simulink model "fix_Current_sync"  (R2025b)
settings: Solver=FixedStepAuto  StartTime=0.0  StopTime=20  FixedStep=0.001  RelTol=1e-3
values from neighbouring files (symbols this model uses):
  Dm = 1e-3    (= 0.001)    [motor_param.m]
  Ki_s = 0.041    [motor_param.m]
  Kp_s = 0.0014    [motor_param.m]
  Ld = 0.01    [motor_param.m]
  Lq = 0.02    [motor_param.m]
  p = 2    [motor_param.m]
  Phi = 0.1    [motor_param.m]
  Rs = 0.38    [motor_param.m]
libraries: fl_lib x50, nesl_utility x50, ee_lib x15, eeTransforms x10, slpidlib x5
(part 1 of 3)
settings Model: Creator=ZhiyongXu  LastModifiedBy=ZhiyongXu

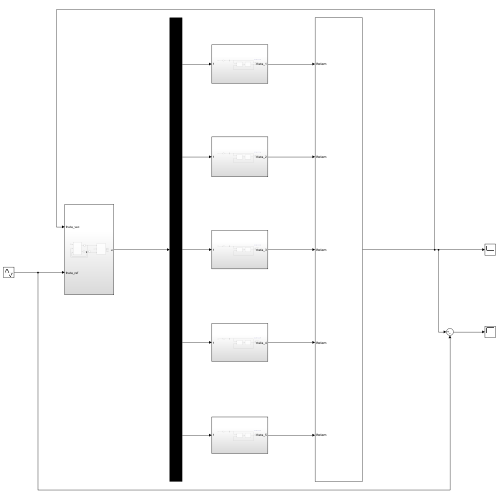
[thumbnail: Simulink's stored preview of the top-level diagram]
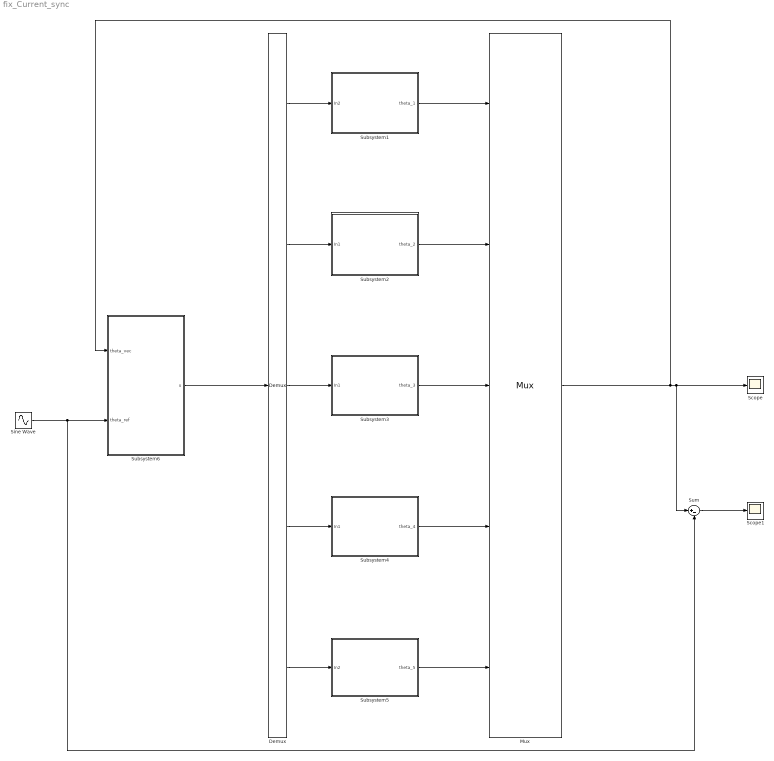
== system fix_Current_sync ==
  Demux : Demux  Outputs=5
  Mux : Mux  Inputs=5
      settings: DisplayOption=signals
  Scope : Scope
      settings: ActiveDisplayYMinimum=-15.273107398212424  ActiveDisplayYMaximum=29.223277886779115  DataLoggingVariableName=ScopeData2  DataLoggingSaveFormat=Array
  Scope1 : Scope
      settings: ActiveDisplayYMinimum=-22.387708842916332  ActiveDisplayYMaximum=22.665034162770731  DataLoggingVariableName=ScopeData3
  Sine Wave : Sin  Amplitude=10  SampleTime=0
  Subsystem1 : Subsystem
  Subsystem2 : Subsystem
  Subsystem3 : Subsystem
  Subsystem4 : Subsystem
  Subsystem5 : Subsystem
  Subsystem6 : Subsystem
  Sum : Sum  Inputs=|+-
  wires:
  Sine Wave/1 -> Sum/2, Subsystem6/2(theta_ref)
  Subsystem6/1(u) -> Demux/1
  Demux/1 -> Subsystem1/1(In2)
  Demux/2 -> Subsystem2/1(In1)
  Demux/3 -> Subsystem3/1(In1)
  Demux/4 -> Subsystem4/1(In1)
  Subsystem1/1(theta_1) -> Mux/1
  Subsystem2/1(theta_2) -> Mux/2
  Subsystem3/1(theta_3) -> Mux/3
  Subsystem4/1(theta_4) -> Mux/4
  Subsystem5/1(theta_5) -> Mux/5
  Sum/1 -> Scope1/1
  Mux/1 -> Sum/1, Scope/1, Subsystem6/1(theta_vec)
  Demux/5 -> Subsystem5/1(In2)

== system fix_Current_sync/Subsystem1 ==
  note: Tune the PI gains of velocity controller
  note: Final Values
  note: Start Values
  In2 : Inport
  Bus Creator : BusCreator  Inputs=1
  Controller : Subsystem
  Evaluation : Subsystem
  Plant : Subsystem
  rpm2rads : Gain
  theta_1 : Outport
  wires:
  Evaluation/1(Out1) -> theta_1/1
  Plant/1(MeasSigs) -> Evaluation/2(MeasSigs), Controller/2(MeasSigs)
  Controller/1(MotCmds) -> Plant/1(MotCmds)
  Bus Creator/1 -> Evaluation/1(TestSigs), Controller/1(TestSigs)
  In2/1 -> rpm2rads/1
  rpm2rads/1 -> Bus Creator/1  "wmref"

== system fix_Current_sync/Subsystem2 ==
  note: Tune the PI gains of velocity controller
  note: Final Values
  note: Start Values
  In1 : Inport
  Bus Creator : BusCreator  Inputs=1
  Controller : Subsystem
  Evaluation : Subsystem
  Plant : Subsystem
  rpm2rads : Gain
  theta_2 : Outport
  wires:
  Evaluation/1(Out1) -> theta_2/1
  Plant/1(MeasSigs) -> Evaluation/2(MeasSigs), Controller/2(MeasSigs)
  Controller/1(MotCmds) -> Plant/1(MotCmds)
  Bus Creator/1 -> Evaluation/1(TestSigs), Controller/1(TestSigs)
  In1/1 -> rpm2rads/1
  rpm2rads/1 -> Bus Creator/1  "wmref"

== system fix_Current_sync/Subsystem3 ==
  note: Tune the PI gains of velocity controller
  note: Final Values
  note: Start Values
  In1 : Inport
  Bus Creator : BusCreator  Inputs=1
  Controller : Subsystem
  Evaluation : Subsystem
  Plant : Subsystem
  rpm2rads : Gain
  theta_3 : Outport
  wires:
  Evaluation/1(Out1) -> theta_3/1
  Plant/1(MeasSigs) -> Evaluation/2(MeasSigs), Controller/2(MeasSigs)
  Controller/1(MotCmds) -> Plant/1(MotCmds)
  Bus Creator/1 -> Evaluation/1(TestSigs), Controller/1(TestSigs)
  rpm2rads/1 -> Bus Creator/1  "wmref"
  In1/1 -> rpm2rads/1

== system fix_Current_sync/Subsystem4 ==
  note: Tune the PI gains of velocity controller
  note: Final Values
  note: Start Values
  In1 : Inport
  Bus Creator : BusCreator  Inputs=1
  Controller : Subsystem
  Evaluation : Subsystem
  Plant : Subsystem
  rpm2rads : Gain
  theta_4 : Outport
  wires:
  Evaluation/1(Out1) -> theta_4/1
  Plant/1(MeasSigs) -> Evaluation/2(MeasSigs), Controller/2(MeasSigs)
  Controller/1(MotCmds) -> Plant/1(MotCmds)
  Bus Creator/1 -> Evaluation/1(TestSigs), Controller/1(TestSigs)
  rpm2rads/1 -> Bus Creator/1  "wmref"
  In1/1 -> rpm2rads/1

== system fix_Current_sync/Subsystem5 ==
  note: Tune the PI gains of velocity controller
  note: Final Values
  note: Start Values
  In2 : Inport
  Bus Creator : BusCreator  Inputs=1
  Controller : Subsystem
  Evaluation : Subsystem
  Plant : Subsystem
  rpm2rads : Gain
  theta_5 : Outport
  wires:
  Evaluation/1(Out1) -> theta_5/1
  Plant/1(MeasSigs) -> Evaluation/2(MeasSigs), Controller/2(MeasSigs)
  Controller/1(MotCmds) -> Plant/1(MotCmds)
  Bus Creator/1 -> Evaluation/1(TestSigs), Controller/1(TestSigs)
  In2/1 -> rpm2rads/1
  rpm2rads/1 -> Bus Creator/1  "wmref"

== system fix_Current_sync/Subsystem6 ==
  theta_vec : Inport
  theta_ref : Inport  Port=2
  Integrator : Integrator
  Integrator1 : Integrator
  MATLAB Function : MATLAB Function  TreatAsAtomicUnit=on
  MATLAB Function4 : MATLAB Function  TreatAsAtomicUnit=on
  Scope : Scope
      settings: ActiveDisplayYMinimum=-6624.1594678331894  ActiveDisplayYMaximum=6466.1304904081144  DataLoggingVariableName=ScopeData4
  Scope1 : Scope
      settings: ActiveDisplayYMinimum=-12.471784481812829  ActiveDisplayYMaximum=55.255314336175005  DataLoggingVariableName=ScopeData5
  u : Outport
  wires:
  MATLAB Function4/1(dth_hat) -> Integrator/1
  MATLAB Function4/2(dom_hat) -> Integrator1/1
  theta_vec/1 -> MATLAB Function/2(theta_meas)
  theta_ref/1 -> MATLAB Function4/1(theta0)
  Integrator1/1 -> Scope1/1, MATLAB Function4/3(om_hat), MATLAB Function/3(om_hat)
  Integrator/1 -> MATLAB Function/1(theta0), MATLAB Function4/2(th_hat)
  MATLAB Function/1(omega_cmd) -> u/1, Scope/1

== system fix_Current_sync/Subsystem1/Controller ==
  TestSigs : Inport
  MeasSigs : Inport  Port=2
  DriverPeripherals : Subsystem
  FOC : Subsystem
  SensorPeripherals : Subsystem
  TestChannel : Subsystem
  MotCmds : Outport  VectorParamsAs1DForOutWhenUnconnected=off
  wires:
  FOC/1(Vabc) -> DriverPeripherals/1(Vabc)
  DriverPeripherals/1(MotCmds) -> MotCmds/1
  TestSigs/1 -> TestChannel/1(TestSigs)
  TestChannel/1(wmref) -> FOC/1(wmref)
  MeasSigs/1 -> SensorPeripherals/1(MeasSigs)
  SensorPeripherals/1(wm) -> FOC/2(wm)
  SensorPeripherals/2(Iabc) -> FOC/3(Iabc)
  SensorPeripherals/3(thetam) -> FOC/4(thetam)

== system fix_Current_sync/Subsystem1/Evaluation ==
  TestSigs : Inport
  MeasSigs : Inport  Port=2
  Bus Selector : BusSelector  OutputSignals=wmref
  Bus Selector1 : BusSelector  OutputSignals=wm,thetam
  Mux : Mux  Inputs=2
  Scope : Scope
      settings: ActiveDisplayYMinimum=-145.10741516627655  ActiveDisplayYMaximum=117.27907525237589
  rads2rpm : Gain
  Out1 : Outport
  wires:
  TestSigs/1 -> Bus Selector/1
  Mux/1 -> rads2rpm/1
  rads2rpm/1 -> Scope/1
  MeasSigs/1 -> Bus Selector1/1
  Bus Selector/1 -> Mux/1  "<wmref>"
  Bus Selector1/2 -> Out1/1  "<thetam>"
  Bus Selector1/1 -> Mux/2  "<wm>"

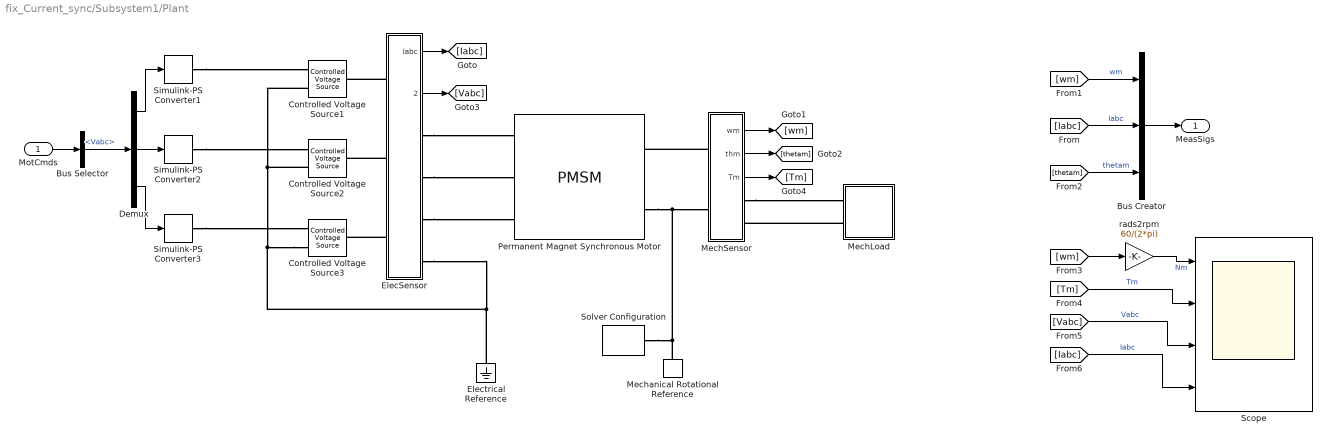
== system fix_Current_sync/Subsystem1/Plant ==
  MotCmds : Inport
  Bus Creator : BusCreator  Inputs=3
  Bus Selector : BusSelector  OutputSignals=Vabc
  Controlled Voltage Source1 : fl_lib/Electrical/Electrical Sources/Controlled Voltage Source
  Controlled Voltage Source2 : fl_lib/Electrical/Electrical Sources/Controlled Voltage Source
  Controlled Voltage Source3 : fl_lib/Electrical/Electrical Sources/Controlled Voltage Source
  Demux : Demux  Outputs=3
  ElecSensor : Subsystem
  Electrical Reference : fl_lib/Electrical/Electrical Elements/Electrical Reference
  MechLoad : Subsystem
  MechSensor : Subsystem
  Mechanical Rotational Reference : fl_lib/Mechanical/Rotational Elements/Mechanical Rotational Reference
  Permanent Magnet Synchronous Motor : ee_lib/Electromechanical/Permanent Magnet/PMSM  port_option=ee.enum.threePhasePort.expanded  winding_type=ee.enum.statorconnection.wye  machine_param=ee.enum.pmsm.parameterization.constant  nPolePairs=p  pmflux_param=1  pm_flux_linkage=Phi Wb  torque_constant=0.18 N*m/A  back_emf_constant=0.18 V/(rad/s)  stator_param=1  Ld=Ld H  Lq=Lq H  idVec=[-200, 0, 200] A  iqVec=[-200, 0, 200] A  LdMatrix=0.0002 * ones(3, 3) H  LqMatrix=0.0002 * ones(3, 3) H  PmMatrix=0.1 * ones(3, 3) Wb  ktMatrix=0.18 * ones(3, 3) N*m/A  keMatrix=0.18 * ones(3, 3) V/(rad/s)  L0=0 H  Ls=0.0002 H  Lm=-0.00002 H  Ms=0.00002 H  Rs=Rs Ohm  zero_sequence=ee.enum.park.zerosequence.exclude  axes_param=2  loss_param=ee.enum.ironloss.none  losses_oc=[0, 0, 0] W  losses_sc=[0, 0, 0] W  f_losses=60 Hz  Isc_losses=95 A  J=0 kg*m^2  lam=0 N*m/(rad/s)  i_d_specify=off  i_d_priority=None  i_d=0 A  i_d_nominal_specify=off  i_d_nominal_value=1  i_d_nominal_unit=A  i_q_specify=off  i_q_priority=None  i_q=0 A  i_q_nominal_specify=off  i_q_nominal_value=1  i_q_nominal_unit=A  torque_specify=off  torque_priority=None  torque=0 N*m  torque_nominal_specify=off  torque_nominal_value=1  torque_nominal_unit=N*m  angular_velocity_specify=on  angular_velocity_priority=High  angular_velocity=100 rpm  angular_velocity_nominal_specify=off  angular_velocity_nominal_value=1  angular_velocity_nominal_unit=rpm  angular_position_specify=off  angular_position_priority=High  angular_position=-2 rad  angular_position_nominal_specify=on  angular_position_nominal_value=100  angular_position_nominal_unit=deg  alpha=3.93e-3 1/K  alpha_flux=-0.001 1/K  Tmeas=298.15 K  stator_thermal_mass=100 J/K  rotor_thermal_mass=200 J/K  Rm_percent_rotor=90  Rd_percent_rotor=30  temperatureA_specify=off  temperatureA_priority=High  temperatureA=25 degC  temperatureA_nominal_specify=off  temperatureA_nominal_value=1  temperatureA_nominal_unit=degC  temperatureB_specify=off  temperatureB_priority=High  temperatureB=25 degC  temperatureB_nominal_specify=off  temperatureB_nominal_value=1  temperatureB_nominal_unit=degC  temperatureC_specify=off  temperatureC_priority=High  temperatureC=25 degC  temperatureC_nominal_specify=off  temperatureC_nominal_value=1  temperatureC_nominal_unit=degC  temperatureR_specify=off  temperatureR_priority=High  temperatureR=25 degC  temperatureR_nominal_specify=off  temperatureR_nominal_value=1  temperatureR_nominal_unit=degC
      settings: InternalSimscapePortConfiguration="{\"Bottom\":[],\"Left\":[{\"id\":\"a\",\"label\":\"a\",\"type\":\"foundation.electrical.electrical\"},{\"id\":\"b\",\"label\":\"b\",\"type\":\"foundation.electrical.electrical\"},{\"id\":\"c\",\"label\":\"c\",\"type\":\"foundation.electrical.electrical\"}],\"Right\":[{\"id\":\"R\",\"label\":\"R\",\"type\":\"foundation.mechanical.rotational.rotational\"},{\"id\":\"C\",\"label\":\"C\",\"type\":\"foundation.mechanical.rotational.rotational\"}],\"Top\":[]}"
  Scope : Scope  NumInputPorts=4
      settings: ActiveDisplayYMinimum=-41.571881527441555  ActiveDisplayYMaximum=115.73020905860461
  Simulink-PS Converter1 : nesl_utility/Simulink-PS Converter  PhysicalDomain=network_engine_domain  SubClassName=ps_input  LeftPortType=input  RightPortType=output  PseudoPeriodic=off  Frequencies=[]  NoiseDistribution=none  NoiseParameters=[]  Unit=1  AffineConversion=off  FilteringAndDerivatives=provide  SimscapeFilterOrder=1  InputFilterTimeConstant=1e-6  UdotUserProvided=0
  Simulink-PS Converter2 : nesl_utility/Simulink-PS Converter  PhysicalDomain=network_engine_domain  SubClassName=ps_input  LeftPortType=input  RightPortType=output  PseudoPeriodic=off  Frequencies=[]  NoiseDistribution=none  NoiseParameters=[]  Unit=1  AffineConversion=off  FilteringAndDerivatives=provide  SimscapeFilterOrder=1  InputFilterTimeConstant=1e-6  UdotUserProvided=0
  Simulink-PS Converter3 : nesl_utility/Simulink-PS Converter  PhysicalDomain=network_engine_domain  SubClassName=ps_input  LeftPortType=input  RightPortType=output  PseudoPeriodic=off  Frequencies=[]  NoiseDistribution=none  NoiseParameters=[]  Unit=1  AffineConversion=off  FilteringAndDerivatives=provide  SimscapeFilterOrder=1  InputFilterTimeConstant=1e-6  UdotUserProvided=0
  Solver Configuration : nesl_utility/Solver Configuration  PhysicalDomain=network_engine_domain  SubClassName=solver  LeftPortType=input  RightPortType=generic  Tones=[]  Harmonics=[]  SimulateNoise=off  Profile=off  UseLocalSampling=off  EnableSwitchedLinearOptims=on  FrequencyDomain=off  UseCCode=off  RelTol=0.001  AbsTol=1e-06  MinStep=1e-09  ToWorkspace=off  RevertToSquareIcSolve=off  NumHomotopyIterations=100  PhasorMode=off  PhasorModeNumHarmonics=1  ConsistencySolver=NEWTON_XTOL_AFTER_FTOL  IndexReductionMethod=DerivativeReplacement  DoDC=off  ResidualTolerance=1e-09  ConsistencyTolSource=GLOBAL  ConsistencyAbsTol=0.001  ConsistencyRelTol=0.001  ConsistencyTolFactor=0.001  UseLocalSolver=off  LocalSolverChoice=NE_BACKWARD_EULER_ADVANCER  ResolveIndetEquations=on  FunctionEvalNumThread=1  LocalSolverSampleTime=0.001  DoFixedCost=off  MaxNonlinIter=3  MaxModeIter=2  ComputeImpulses=off  ImpulseIterations=2  LinearAlgebra=Sparse  LinearAlgebraNumThread=0  EquationFormulation=NE_TIME_EF  DelaysMemoryBudget=1024  AutomaticFiltering=on  FilteringTimeConstant=0.001  PartitionStorageMethod=AS_NEEDED  PartitionMemoryBudget=1024  PartitionMethod=FAST  MultibodyUseLocalSolver=off  MultibodyLocalSolverChoice=ODE1  MultibodyLocalSolverSampleTime=0.001
  rads2rpm : Gain  Gain=60/(2*pi)
  MeasSigs : Outport  VectorParamsAs1DForOutWhenUnconnected=off
  wires:
  ElecSensor/1(Iabc) -> [Iabc]
  ElecSensor/2(Vabc) -> [Vabc]
  Demux/2 -> Simulink-PS Converter2/1
  Demux/1 -> Simulink-PS Converter1/1
  Demux/3 -> Simulink-PS Converter3/1
  MechSensor/1(wm) -> [wm]
  MechSensor/2(thm) -> [thetam]
  MechSensor/3(Tm) -> [Tm]
  [wm] -> Bus Creator/1  "wm"
  [Iabc] -> Bus Creator/2  "Iabc"
  [thetam] -> Bus Creator/3  "thetam"
  Bus Creator/1 -> MeasSigs/1
  MotCmds/1 -> Bus Selector/1
  Bus Selector/1 -> Demux/1  "<Vabc>"
  [wm] -> rads2rpm/1
  rads2rpm/1 -> Scope/1  "Nm"
  [Tm] -> Scope/2  "Tm"
  [Vabc] -> Scope/3  "Vabc"
  [Iabc] -> Scope/4  "Iabc"
  connections:
  Simulink-PS Converter2/RConn1 -- Controlled Voltage Source2/RConn1
  Simulink-PS Converter3/RConn1 -- Controlled Voltage Source3/RConn1
  ElecSensor/RConn3 -- Permanent Magnet Synchronous Motor/LConn3
  ElecSensor/LConn2 -- Controlled Voltage Source2/LConn1
  Controlled Voltage Source3/RConn2 -- Controlled Voltage Source1/RConn2 -- Controlled Voltage Source2/RConn2 -- ElecSensor/RConn4 -- Electrical Reference/LConn1
  ElecSensor/RConn2 -- Permanent Magnet Synchronous Motor/LConn2
  ElecSensor/RConn1 -- Permanent Magnet Synchronous Motor/LConn1
  ElecSensor/LConn3 -- Controlled Voltage Source3/LConn1
  ElecSensor/LConn1 -- Controlled Voltage Source1/LConn1
  Simulink-PS Converter1/RConn1 -- Controlled Voltage Source1/RConn1
  Permanent Magnet Synchronous Motor/RConn2 -- Solver Configuration/RConn1 -- Mechanical Rotational Reference/LConn1 -- MechSensor/LConn2
  MechSensor/RConn1 -- MechLoad/LConn1
  MechLoad/LConn2 -- MechSensor/RConn2
  MechSensor/LConn1 -- Permanent Magnet Synchronous Motor/RConn1

== system fix_Current_sync/Subsystem2/Controller ==
  TestSigs : Inport
  MeasSigs : Inport  Port=2
  DriverPeripherals : Subsystem
  FOC : Subsystem
  SensorPeripherals : Subsystem
  TestChannel : Subsystem
  MotCmds : Outport  VectorParamsAs1DForOutWhenUnconnected=off
  wires:
  FOC/1(Vabc) -> DriverPeripherals/1(Vabc)
  DriverPeripherals/1(MotCmds) -> MotCmds/1
  TestSigs/1 -> TestChannel/1(TestSigs)
  TestChannel/1(wmref) -> FOC/1(wmref)
  MeasSigs/1 -> SensorPeripherals/1(MeasSigs)
  SensorPeripherals/1(wm) -> FOC/2(wm)
  SensorPeripherals/2(Iabc) -> FOC/3(Iabc)
  SensorPeripherals/3(thetam) -> FOC/4(thetam)

== system fix_Current_sync/Subsystem2/Evaluation ==
  TestSigs : Inport
  MeasSigs : Inport  Port=2
  Bus Selector : BusSelector  OutputSignals=wmref
  Bus Selector1 : BusSelector  OutputSignals=wm,thetam
  Mux : Mux  Inputs=2
  Scope : Scope
      settings: ActiveDisplayYMinimum=-28.436313686078961  ActiveDisplayYMaximum=12.340264545018567
  rads2rpm : Gain
  Out1 : Outport
  wires:
  TestSigs/1 -> Bus Selector/1
  Mux/1 -> rads2rpm/1
  rads2rpm/1 -> Scope/1
  MeasSigs/1 -> Bus Selector1/1
  Bus Selector/1 -> Mux/1  "<wmref>"
  Bus Selector1/2 -> Out1/1  "<thetam>"
  Bus Selector1/1 -> Mux/2  "<wm>"

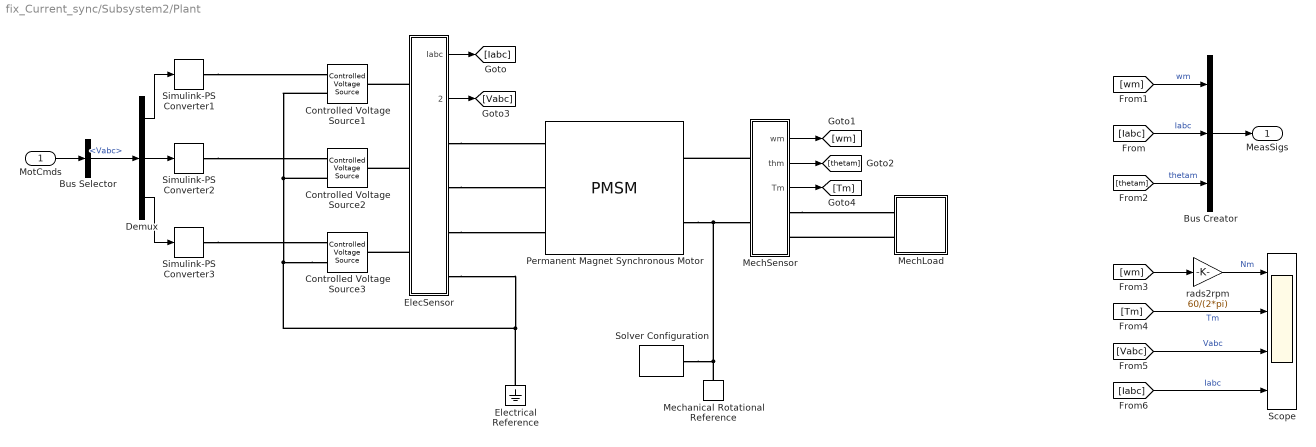
== system fix_Current_sync/Subsystem2/Plant ==
  MotCmds : Inport
  Bus Creator : BusCreator  Inputs=3
  Bus Selector : BusSelector  OutputSignals=Vabc
  Controlled Voltage Source1 : fl_lib/Electrical/Electrical Sources/Controlled Voltage Source
  Controlled Voltage Source2 : fl_lib/Electrical/Electrical Sources/Controlled Voltage Source
  Controlled Voltage Source3 : fl_lib/Electrical/Electrical Sources/Controlled Voltage Source
  Demux : Demux  Outputs=3
  ElecSensor : Subsystem
  Electrical Reference : fl_lib/Electrical/Electrical Elements/Electrical Reference
  MechLoad : Subsystem
  MechSensor : Subsystem
  Mechanical Rotational Reference : fl_lib/Mechanical/Rotational Elements/Mechanical Rotational Reference
  Permanent Magnet Synchronous Motor : ee_lib/Electromechanical/Permanent Magnet/PMSM  port_option=ee.enum.threePhasePort.expanded  winding_type=ee.enum.statorconnection.wye  machine_param=ee.enum.pmsm.parameterization.constant  nPolePairs=p  pmflux_param=1  pm_flux_linkage=Phi Wb  torque_constant=0.18 N*m/A  back_emf_constant=0.18 V/(rad/s)  stator_param=1  Ld=Ld H  Lq=Lq H  idVec=[-200, 0, 200] A  iqVec=[-200, 0, 200] A  LdMatrix=0.0002 * ones(3, 3) H  LqMatrix=0.0002 * ones(3, 3) H  PmMatrix=0.1 * ones(3, 3) Wb  ktMatrix=0.18 * ones(3, 3) N*m/A  keMatrix=0.18 * ones(3, 3) V/(rad/s)  L0=0 H  Ls=0.0002 H  Lm=-0.00002 H  Ms=0.00002 H  Rs=Rs Ohm  zero_sequence=ee.enum.park.zerosequence.exclude  axes_param=2  loss_param=ee.enum.ironloss.none  losses_oc=[0, 0, 0] W  losses_sc=[0, 0, 0] W  f_losses=60 Hz  Isc_losses=95 A  J=0 kg*m^2  lam=0 N*m/(rad/s)  i_d_specify=off  i_d_priority=None  i_d=0 A  i_d_nominal_specify=off  i_d_nominal_value=1  i_d_nominal_unit=A  i_q_specify=off  i_q_priority=None  i_q=0 A  i_q_nominal_specify=off  i_q_nominal_value=1  i_q_nominal_unit=A  torque_specify=off  torque_priority=None  torque=0 N*m  torque_nominal_specify=off  torque_nominal_value=1  torque_nominal_unit=N*m  angular_velocity_specify=on  angular_velocity_priority=High  angular_velocity=50 rpm  angular_velocity_nominal_specify=off  angular_velocity_nominal_value=1  angular_velocity_nominal_unit=rpm  angular_position_specify=on  angular_position_priority=High  angular_position=10 deg  angular_position_nominal_specify=off  angular_position_nominal_value=1  angular_position_nominal_unit=deg  alpha=3.93e-3 1/K  alpha_flux=-0.001 1/K  Tmeas=298.15 K  stator_thermal_mass=100 J/K  rotor_thermal_mass=200 J/K  Rm_percent_rotor=90  Rd_percent_rotor=30  temperatureA_specify=off  temperatureA_priority=High  temperatureA=25 degC  temperatureA_nominal_specify=off  temperatureA_nominal_value=1  temperatureA_nominal_unit=degC  temperatureB_specify=off  temperatureB_priority=High  temperatureB=25 degC  temperatureB_nominal_specify=off  temperatureB_nominal_value=1  temperatureB_nominal_unit=degC  temperatureC_specify=off  temperatureC_priority=High  temperatureC=25 degC  temperatureC_nominal_specify=off  temperatureC_nominal_value=1  temperatureC_nominal_unit=degC  temperatureR_specify=off  temperatureR_priority=High  temperatureR=25 degC  temperatureR_nominal_specify=off  temperatureR_nominal_value=1  temperatureR_nominal_unit=degC
      settings: InternalSimscapePortConfiguration="{\"Bottom\":[],\"Left\":[{\"id\":\"a\",\"label\":\"a\",\"type\":\"foundation.electrical.electrical\"},{\"id\":\"b\",\"label\":\"b\",\"type\":\"foundation.electrical.electrical\"},{\"id\":\"c\",\"label\":\"c\",\"type\":\"foundation.electrical.electrical\"}],\"Right\":[{\"id\":\"R\",\"label\":\"R\",\"type\":\"foundation.mechanical.rotational.rotational\"},{\"id\":\"C\",\"label\":\"C\",\"type\":\"foundation.mechanical.rotational.rotational\"}],\"Top\":[]}"
  Scope : Scope  NumInputPorts=4
      settings: ActiveDisplayYMinimum=-1  ActiveDisplayYMaximum=1
  Simulink-PS Converter1 : nesl_utility/Simulink-PS Converter  PhysicalDomain=network_engine_domain  SubClassName=ps_input  LeftPortType=input  RightPortType=output  PseudoPeriodic=off  Frequencies=[]  NoiseDistribution=none  NoiseParameters=[]  Unit=1  AffineConversion=off  FilteringAndDerivatives=provide  SimscapeFilterOrder=1  InputFilterTimeConstant=1e-6  UdotUserProvided=0
  Simulink-PS Converter2 : nesl_utility/Simulink-PS Converter  PhysicalDomain=network_engine_domain  SubClassName=ps_input  LeftPortType=input  RightPortType=output  PseudoPeriodic=off  Frequencies=[]  NoiseDistribution=none  NoiseParameters=[]  Unit=1  AffineConversion=off  FilteringAndDerivatives=provide  SimscapeFilterOrder=1  InputFilterTimeConstant=1e-6  UdotUserProvided=0
  Simulink-PS Converter3 : nesl_utility/Simulink-PS Converter  PhysicalDomain=network_engine_domain  SubClassName=ps_input  LeftPortType=input  RightPortType=output  PseudoPeriodic=off  Frequencies=[]  NoiseDistribution=none  NoiseParameters=[]  Unit=1  AffineConversion=off  FilteringAndDerivatives=provide  SimscapeFilterOrder=1  InputFilterTimeConstant=1e-6  UdotUserProvided=0
  Solver Configuration : nesl_utility/Solver Configuration  PhysicalDomain=network_engine_domain  SubClassName=solver  LeftPortType=input  RightPortType=generic  Tones=[]  Harmonics=[]  SimulateNoise=off  Profile=off  UseLocalSampling=off  EnableSwitchedLinearOptims=on  FrequencyDomain=off  UseCCode=off  RelTol=0.001  AbsTol=1e-06  MinStep=1e-09  ToWorkspace=off  RevertToSquareIcSolve=off  NumHomotopyIterations=100  PhasorMode=off  PhasorModeNumHarmonics=1  ConsistencySolver=NEWTON_XTOL_AFTER_FTOL  IndexReductionMethod=DerivativeReplacement  DoDC=off  ResidualTolerance=1e-09  ConsistencyTolSource=GLOBAL  ConsistencyAbsTol=0.001  ConsistencyRelTol=0.001  ConsistencyTolFactor=0.001  UseLocalSolver=off  LocalSolverChoice=NE_BACKWARD_EULER_ADVANCER  ResolveIndetEquations=on  FunctionEvalNumThread=1  LocalSolverSampleTime=0.001  DoFixedCost=off  MaxNonlinIter=3  MaxModeIter=2  ComputeImpulses=off  ImpulseIterations=2  LinearAlgebra=Sparse  LinearAlgebraNumThread=0  EquationFormulation=NE_TIME_EF  DelaysMemoryBudget=1024  AutomaticFiltering=on  FilteringTimeConstant=0.001  PartitionStorageMethod=AS_NEEDED  PartitionMemoryBudget=1024  PartitionMethod=FAST  MultibodyUseLocalSolver=off  MultibodyLocalSolverChoice=ODE1  MultibodyLocalSolverSampleTime=0.001
  rads2rpm : Gain  Gain=60/(2*pi)
  MeasSigs : Outport  VectorParamsAs1DForOutWhenUnconnected=off
  wires:
  ElecSensor/1(Iabc) -> [Iabc]
  ElecSensor/2(Vabc) -> [Vabc]
  Demux/2 -> Simulink-PS Converter2/1
  Demux/1 -> Simulink-PS Converter1/1
  Demux/3 -> Simulink-PS Converter3/1
  MechSensor/1(wm) -> [wm]
  MechSensor/2(thm) -> [thetam]
  MechSensor/3(Tm) -> [Tm]
  [wm] -> Bus Creator/1  "wm"
  [Iabc] -> Bus Creator/2  "Iabc"
  [thetam] -> Bus Creator/3  "thetam"
  Bus Creator/1 -> MeasSigs/1
  MotCmds/1 -> Bus Selector/1
  Bus Selector/1 -> Demux/1  "<Vabc>"
  [wm] -> rads2rpm/1
  rads2rpm/1 -> Scope/1  "Nm"
  [Tm] -> Scope/2  "Tm"
  [Vabc] -> Scope/3  "Vabc"
  [Iabc] -> Scope/4  "Iabc"
  connections:
  Simulink-PS Converter2/RConn1 -- Controlled Voltage Source2/RConn1
  Simulink-PS Converter3/RConn1 -- Controlled Voltage Source3/RConn1
  ElecSensor/RConn3 -- Permanent Magnet Synchronous Motor/LConn3
  ElecSensor/LConn2 -- Controlled Voltage Source2/LConn1
  Controlled Voltage Source3/RConn2 -- Controlled Voltage Source1/RConn2 -- Controlled Voltage Source2/RConn2 -- ElecSensor/RConn4 -- Electrical Reference/LConn1
  ElecSensor/RConn2 -- Permanent Magnet Synchronous Motor/LConn2
  ElecSensor/RConn1 -- Permanent Magnet Synchronous Motor/LConn1
  ElecSensor/LConn3 -- Controlled Voltage Source3/LConn1
  ElecSensor/LConn1 -- Controlled Voltage Source1/LConn1
  Simulink-PS Converter1/RConn1 -- Controlled Voltage Source1/RConn1
  Permanent Magnet Synchronous Motor/RConn2 -- Solver Configuration/RConn1 -- Mechanical Rotational Reference/LConn1 -- MechSensor/LConn2
  MechSensor/RConn1 -- MechLoad/LConn1
  MechLoad/LConn2 -- MechSensor/RConn2
  MechSensor/LConn1 -- Permanent Magnet Synchronous Motor/RConn1

== system fix_Current_sync/Subsystem3/Controller ==
  TestSigs : Inport
  MeasSigs : Inport  Port=2
  DriverPeripherals : Subsystem
  FOC : Subsystem
  SensorPeripherals : Subsystem
  TestChannel : Subsystem
  MotCmds : Outport  VectorParamsAs1DForOutWhenUnconnected=off
  wires:
  FOC/1(Vabc) -> DriverPeripherals/1(Vabc)
  DriverPeripherals/1(MotCmds) -> MotCmds/1
  TestSigs/1 -> TestChannel/1(TestSigs)
  TestChannel/1(wmref) -> FOC/1(wmref)
  MeasSigs/1 -> SensorPeripherals/1(MeasSigs)
  SensorPeripherals/1(wm) -> FOC/2(wm)
  SensorPeripherals/2(Iabc) -> FOC/3(Iabc)
  SensorPeripherals/3(thetam) -> FOC/4(thetam)

== system fix_Current_sync/Subsystem3/Evaluation ==
  TestSigs : Inport
  MeasSigs : Inport  Port=2
  Bus Selector : BusSelector  OutputSignals=wmref
  Bus Selector1 : BusSelector  OutputSignals=wm,thetam
  Mux : Mux  Inputs=2
  Scope : Scope
      settings: ActiveDisplayYMinimum=-3107.1721459970354  ActiveDisplayYMaximum=3159.6442979714316
  rads2rpm : Gain
  Out1 : Outport
  wires:
  TestSigs/1 -> Bus Selector/1
  Mux/1 -> rads2rpm/1
  rads2rpm/1 -> Scope/1
  MeasSigs/1 -> Bus Selector1/1
  Bus Selector/1 -> Mux/1  "<wmref>"
  Bus Selector1/1 -> Mux/2  "<wm>"
  Bus Selector1/2 -> Out1/1  "<thetam>"

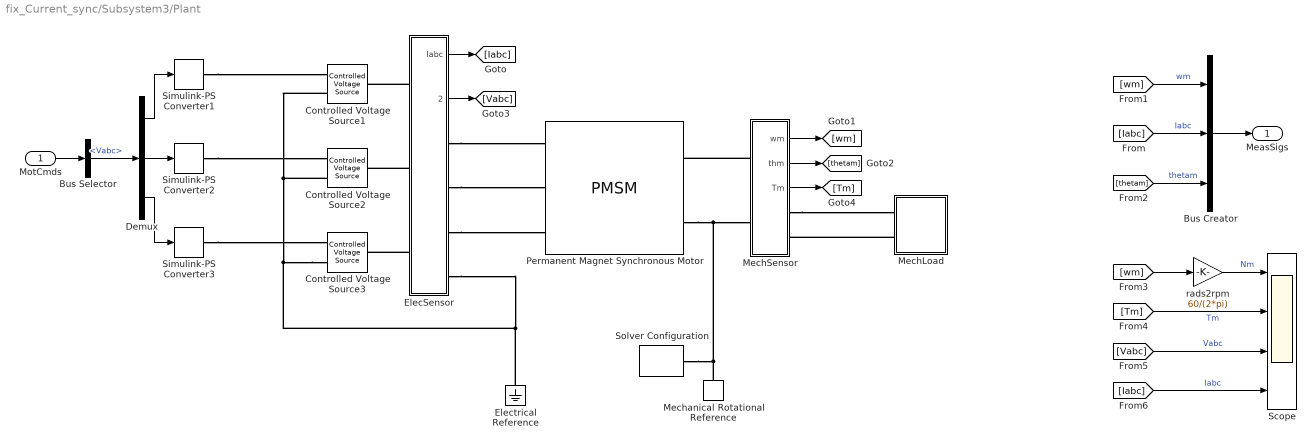
== system fix_Current_sync/Subsystem3/Plant ==
  MotCmds : Inport
  Bus Creator : BusCreator  Inputs=3
  Bus Selector : BusSelector  OutputSignals=Vabc
  Controlled Voltage Source1 : fl_lib/Electrical/Electrical Sources/Controlled Voltage Source
  Controlled Voltage Source2 : fl_lib/Electrical/Electrical Sources/Controlled Voltage Source
  Controlled Voltage Source3 : fl_lib/Electrical/Electrical Sources/Controlled Voltage Source
  Demux : Demux  Outputs=3
  ElecSensor : Subsystem
  Electrical Reference : fl_lib/Electrical/Electrical Elements/Electrical Reference
  MechLoad : Subsystem
  MechSensor : Subsystem
  Mechanical Rotational Reference : fl_lib/Mechanical/Rotational Elements/Mechanical Rotational Reference
  Permanent Magnet Synchronous Motor : ee_lib/Electromechanical/Permanent Magnet/PMSM  port_option=ee.enum.threePhasePort.expanded  winding_type=ee.enum.statorconnection.wye  machine_param=ee.enum.pmsm.parameterization.constant  nPolePairs=p  pmflux_param=1  pm_flux_linkage=Phi Wb  torque_constant=0.18 N*m/A  back_emf_constant=0.18 V/(rad/s)  stator_param=1  Ld=Ld H  Lq=Lq H  idVec=[-200, 0, 200] A  iqVec=[-200, 0, 200] A  LdMatrix=0.0002 * ones(3, 3) H  LqMatrix=0.0002 * ones(3, 3) H  PmMatrix=0.1 * ones(3, 3) Wb  ktMatrix=0.18 * ones(3, 3) N*m/A  keMatrix=0.18 * ones(3, 3) V/(rad/s)  L0=0 H  Ls=0.0002 H  Lm=-0.00002 H  Ms=0.00002 H  Rs=Rs Ohm  zero_sequence=ee.enum.park.zerosequence.exclude  axes_param=2  loss_param=ee.enum.ironloss.none  losses_oc=[0, 0, 0] W  losses_sc=[0, 0, 0] W  f_losses=60 Hz  Isc_losses=95 A  J=0 kg*m^2  lam=0 N*m/(rad/s)  i_d_specify=off  i_d_priority=None  i_d=0 A  i_d_nominal_specify=off  i_d_nominal_value=1  i_d_nominal_unit=A  i_q_specify=off  i_q_priority=None  i_q=0 A  i_q_nominal_specify=off  i_q_nominal_value=1  i_q_nominal_unit=A  torque_specify=off  torque_priority=None  torque=0 N*m  torque_nominal_specify=off  torque_nominal_value=1  torque_nominal_unit=N*m  angular_velocity_specify=on  angular_velocity_priority=High  angular_velocity=0 rpm  angular_velocity_nominal_specify=off  angular_velocity_nominal_value=1  angular_velocity_nominal_unit=rpm  angular_position_specify=off  angular_position_priority=High  angular_position=0 deg  angular_position_nominal_specify=off  angular_position_nominal_value=1  angular_position_nominal_unit=deg  alpha=3.93e-3 1/K  alpha_flux=-0.001 1/K  Tmeas=298.15 K  stator_thermal_mass=100 J/K  rotor_thermal_mass=200 J/K  Rm_percent_rotor=90  Rd_percent_rotor=30  temperatureA_specify=off  temperatureA_priority=High  temperatureA=25 degC  temperatureA_nominal_specify=off  temperatureA_nominal_value=1  temperatureA_nominal_unit=degC  temperatureB_specify=off  temperatureB_priority=High  temperatureB=25 degC  temperatureB_nominal_specify=off  temperatureB_nominal_value=1  temperatureB_nominal_unit=degC  temperatureC_specify=off  temperatureC_priority=High  temperatureC=25 degC  temperatureC_nominal_specify=off  temperatureC_nominal_value=1  temperatureC_nominal_unit=degC  temperatureR_specify=off  temperatureR_priority=High  temperatureR=25 degC  temperatureR_nominal_specify=off  temperatureR_nominal_value=1  temperatureR_nominal_unit=degC
      settings: InternalSimscapePortConfiguration="{\"Bottom\":[],\"Left\":[{\"id\":\"a\",\"label\":\"a\",\"type\":\"foundation.electrical.electrical\"},{\"id\":\"b\",\"label\":\"b\",\"type\":\"foundation.electrical.electrical\"},{\"id\":\"c\",\"label\":\"c\",\"type\":\"foundation.electrical.electrical\"}],\"Right\":[{\"id\":\"R\",\"label\":\"R\",\"type\":\"foundation.mechanical.rotational.rotational\"},{\"id\":\"C\",\"label\":\"C\",\"type\":\"foundation.mechanical.rotational.rotational\"}],\"Top\":[]}"
  Scope : Scope  NumInputPorts=4
      settings: ActiveDisplayYMinimum=-2500.2768341970282  ActiveDisplayYMaximum=2500.1048598569782
  Simulink-PS Converter1 : nesl_utility/Simulink-PS Converter  PhysicalDomain=network_engine_domain  SubClassName=ps_input  LeftPortType=input  RightPortType=output  PseudoPeriodic=off  Frequencies=[]  NoiseDistribution=none  NoiseParameters=[]  Unit=1  AffineConversion=off  FilteringAndDerivatives=provide  SimscapeFilterOrder=1  InputFilterTimeConstant=1e-6  UdotUserProvided=0
  Simulink-PS Converter2 : nesl_utility/Simulink-PS Converter  PhysicalDomain=network_engine_domain  SubClassName=ps_input  LeftPortType=input  RightPortType=output  PseudoPeriodic=off  Frequencies=[]  NoiseDistribution=none  NoiseParameters=[]  Unit=1  AffineConversion=off  FilteringAndDerivatives=provide  SimscapeFilterOrder=1  InputFilterTimeConstant=1e-6  UdotUserProvided=0
  Simulink-PS Converter3 : nesl_utility/Simulink-PS Converter  PhysicalDomain=network_engine_domain  SubClassName=ps_input  LeftPortType=input  RightPortType=output  PseudoPeriodic=off  Frequencies=[]  NoiseDistribution=none  NoiseParameters=[]  Unit=1  AffineConversion=off  FilteringAndDerivatives=provide  SimscapeFilterOrder=1  InputFilterTimeConstant=1e-6  UdotUserProvided=0
  Solver Configuration : nesl_utility/Solver Configuration  PhysicalDomain=network_engine_domain  SubClassName=solver  LeftPortType=input  RightPortType=generic  Tones=[]  Harmonics=[]  SimulateNoise=off  Profile=off  UseLocalSampling=off  EnableSwitchedLinearOptims=on  FrequencyDomain=off  UseCCode=off  RelTol=0.001  AbsTol=1e-06  MinStep=1e-09  ToWorkspace=off  RevertToSquareIcSolve=off  NumHomotopyIterations=100  PhasorMode=off  PhasorModeNumHarmonics=1  ConsistencySolver=NEWTON_XTOL_AFTER_FTOL  IndexReductionMethod=DerivativeReplacement  DoDC=off  ResidualTolerance=1e-09  ConsistencyTolSource=GLOBAL  ConsistencyAbsTol=0.001  ConsistencyRelTol=0.001  ConsistencyTolFactor=0.001  UseLocalSolver=off  LocalSolverChoice=NE_BACKWARD_EULER_ADVANCER  ResolveIndetEquations=on  FunctionEvalNumThread=1  LocalSolverSampleTime=0.001  DoFixedCost=off  MaxNonlinIter=3  MaxModeIter=2  ComputeImpulses=off  ImpulseIterations=2  LinearAlgebra=Sparse  LinearAlgebraNumThread=0  EquationFormulation=NE_TIME_EF  DelaysMemoryBudget=1024  AutomaticFiltering=on  FilteringTimeConstant=0.001  PartitionStorageMethod=AS_NEEDED  PartitionMemoryBudget=1024  PartitionMethod=FAST  MultibodyUseLocalSolver=off  MultibodyLocalSolverChoice=ODE1  MultibodyLocalSolverSampleTime=0.001
  rads2rpm : Gain  Gain=60/(2*pi)
  MeasSigs : Outport  VectorParamsAs1DForOutWhenUnconnected=off
  wires:
  ElecSensor/1(Iabc) -> [Iabc]
  ElecSensor/2(Vabc) -> [Vabc]
  Demux/2 -> Simulink-PS Converter2/1
  Demux/1 -> Simulink-PS Converter1/1
  Demux/3 -> Simulink-PS Converter3/1
  MechSensor/1(wm) -> [wm]
  MechSensor/2(thm) -> [thetam]
  MechSensor/3(Tm) -> [Tm]
  [wm] -> Bus Creator/1  "wm"
  [Iabc] -> Bus Creator/2  "Iabc"
  [thetam] -> Bus Creator/3  "thetam"
  Bus Creator/1 -> MeasSigs/1
  MotCmds/1 -> Bus Selector/1
  Bus Selector/1 -> Demux/1  "<Vabc>"
  [wm] -> rads2rpm/1
  rads2rpm/1 -> Scope/1  "Nm"
  [Tm] -> Scope/2  "Tm"
  [Vabc] -> Scope/3  "Vabc"
  [Iabc] -> Scope/4  "Iabc"
  connections:
  Simulink-PS Converter2/RConn1 -- Controlled Voltage Source2/RConn1
  Simulink-PS Converter3/RConn1 -- Controlled Voltage Source3/RConn1
  ElecSensor/RConn3 -- Permanent Magnet Synchronous Motor/LConn3
  ElecSensor/LConn2 -- Controlled Voltage Source2/LConn1
  Controlled Voltage Source3/RConn2 -- Controlled Voltage Source1/RConn2 -- Controlled Voltage Source2/RConn2 -- ElecSensor/RConn4 -- Electrical Reference/LConn1
  ElecSensor/RConn2 -- Permanent Magnet Synchronous Motor/LConn2
  ElecSensor/RConn1 -- Permanent Magnet Synchronous Motor/LConn1
  ElecSensor/LConn3 -- Controlled Voltage Source3/LConn1
  ElecSensor/LConn1 -- Controlled Voltage Source1/LConn1
  Simulink-PS Converter1/RConn1 -- Controlled Voltage Source1/RConn1
  Permanent Magnet Synchronous Motor/RConn2 -- Solver Configuration/RConn1 -- Mechanical Rotational Reference/LConn1 -- MechSensor/LConn2
  MechSensor/RConn1 -- MechLoad/LConn1
  MechLoad/LConn2 -- MechSensor/RConn2
  MechSensor/LConn1 -- Permanent Magnet Synchronous Motor/RConn1

== system fix_Current_sync/Subsystem4/Controller ==
  TestSigs : Inport
  MeasSigs : Inport  Port=2
  DriverPeripherals : Subsystem
  FOC : Subsystem
  SensorPeripherals : Subsystem
  TestChannel : Subsystem
  MotCmds : Outport  VectorParamsAs1DForOutWhenUnconnected=off
  wires:
  FOC/1(Vabc) -> DriverPeripherals/1(Vabc)
  DriverPeripherals/1(MotCmds) -> MotCmds/1
  TestSigs/1 -> TestChannel/1(TestSigs)
  TestChannel/1(wmref) -> FOC/1(wmref)
  MeasSigs/1 -> SensorPeripherals/1(MeasSigs)
  SensorPeripherals/1(wm) -> FOC/2(wm)
  SensorPeripherals/2(Iabc) -> FOC/3(Iabc)
  SensorPeripherals/3(thetam) -> FOC/4(thetam)

== system fix_Current_sync/Subsystem4/Evaluation ==
  TestSigs : Inport
  MeasSigs : Inport  Port=2
  Bus Selector : BusSelector  OutputSignals=wmref
  Bus Selector1 : BusSelector  OutputSignals=wm,thetam
  Mux : Mux  Inputs=2
  Scope : Scope
      settings: ActiveDisplayYMinimum=-3107.1721459970354  ActiveDisplayYMaximum=3159.6442979714316
  rads2rpm : Gain
  Out1 : Outport
  wires:
  TestSigs/1 -> Bus Selector/1
  Mux/1 -> rads2rpm/1
  rads2rpm/1 -> Scope/1
  MeasSigs/1 -> Bus Selector1/1
  Bus Selector/1 -> Mux/1  "<wmref>"
  Bus Selector1/1 -> Mux/2  "<wm>"
  Bus Selector1/2 -> Out1/1  "<thetam>"

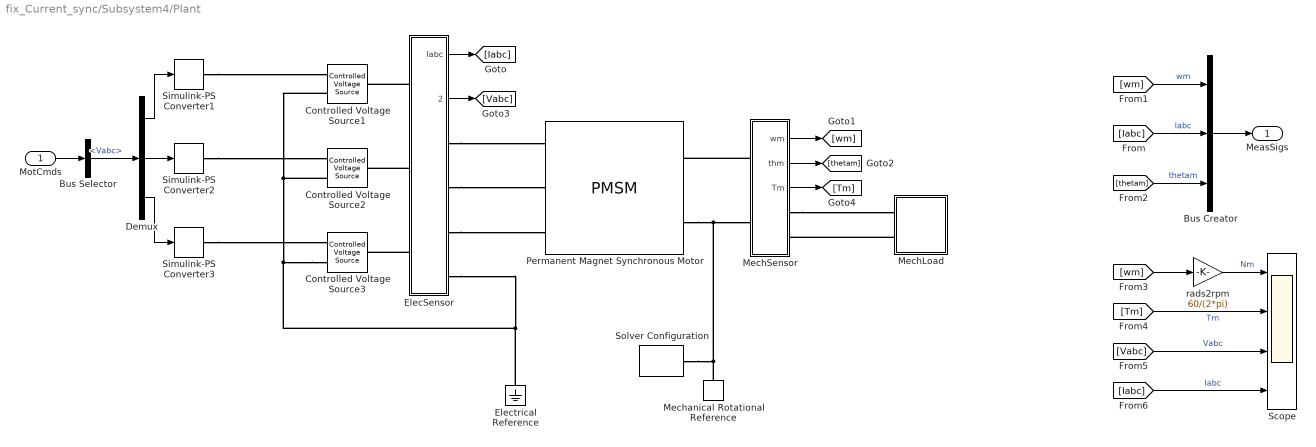
== system fix_Current_sync/Subsystem4/Plant ==
  MotCmds : Inport
  Bus Creator : BusCreator  Inputs=3
  Bus Selector : BusSelector  OutputSignals=Vabc
  Controlled Voltage Source1 : fl_lib/Electrical/Electrical Sources/Controlled Voltage Source
  Controlled Voltage Source2 : fl_lib/Electrical/Electrical Sources/Controlled Voltage Source
  Controlled Voltage Source3 : fl_lib/Electrical/Electrical Sources/Controlled Voltage Source
  Demux : Demux  Outputs=3
  ElecSensor : Subsystem
  Electrical Reference : fl_lib/Electrical/Electrical Elements/Electrical Reference
  MechLoad : Subsystem
  MechSensor : Subsystem
  Mechanical Rotational Reference : fl_lib/Mechanical/Rotational Elements/Mechanical Rotational Reference
  Permanent Magnet Synchronous Motor : ee_lib/Electromechanical/Permanent Magnet/PMSM  port_option=ee.enum.threePhasePort.expanded  winding_type=ee.enum.statorconnection.wye  machine_param=ee.enum.pmsm.parameterization.constant  nPolePairs=p  pmflux_param=1  pm_flux_linkage=Phi Wb  torque_constant=0.18 N*m/A  back_emf_constant=0.18 V/(rad/s)  stator_param=1  Ld=Ld H  Lq=Lq H  idVec=[-200, 0, 200] A  iqVec=[-200, 0, 200] A  LdMatrix=0.0002 * ones(3, 3) H  LqMatrix=0.0002 * ones(3, 3) H  PmMatrix=0.1 * ones(3, 3) Wb  ktMatrix=0.18 * ones(3, 3) N*m/A  keMatrix=0.18 * ones(3, 3) V/(rad/s)  L0=0 H  Ls=0.0002 H  Lm=-0.00002 H  Ms=0.00002 H  Rs=Rs Ohm  zero_sequence=ee.enum.park.zerosequence.exclude  axes_param=2  loss_param=ee.enum.ironloss.none  losses_oc=[0, 0, 0] W  losses_sc=[0, 0, 0] W  f_losses=60 Hz  Isc_losses=95 A  J=0 kg*m^2  lam=0 N*m/(rad/s)  i_d_specify=off  i_d_priority=None  i_d=0 A  i_d_nominal_specify=off  i_d_nominal_value=1  i_d_nominal_unit=A  i_q_specify=off  i_q_priority=None  i_q=0 A  i_q_nominal_specify=off  i_q_nominal_value=1  i_q_nominal_unit=A  torque_specify=off  torque_priority=None  torque=0 N*m  torque_nominal_specify=off  torque_nominal_value=1  torque_nominal_unit=N*m  angular_velocity_specify=off  angular_velocity_priority=High  angular_velocity=-50 rpm  angular_velocity_nominal_specify=off  angular_velocity_nominal_value=1  angular_velocity_nominal_unit=rpm  angular_position_specify=on  angular_position_priority=High  angular_position=-10 deg  angular_position_nominal_specify=on  angular_position_nominal_value=20  angular_position_nominal_unit=deg  alpha=3.93e-3 1/K  alpha_flux=-0.001 1/K  Tmeas=298.15 K  stator_thermal_mass=100 J/K  rotor_thermal_mass=200 J/K  Rm_percent_rotor=90  Rd_percent_rotor=30  temperatureA_specify=off  temperatureA_priority=High  temperatureA=25 degC  temperatureA_nominal_specify=off  temperatureA_nominal_value=1  temperatureA_nominal_unit=degC  temperatureB_specify=off  temperatureB_priority=High  temperatureB=25 degC  temperatureB_nominal_specify=off  temperatureB_nominal_value=1  temperatureB_nominal_unit=degC  temperatureC_specify=off  temperatureC_priority=High  temperatureC=25 degC  temperatureC_nominal_specify=off  temperatureC_nominal_value=1  temperatureC_nominal_unit=degC  temperatureR_specify=off  temperatureR_priority=High  temperatureR=25 degC  temperatureR_nominal_specify=off  temperatureR_nominal_value=1  temperatureR_nominal_unit=degC
      settings: InternalSimscapePortConfiguration="{\"Bottom\":[],\"Left\":[{\"id\":\"a\",\"label\":\"a\",\"type\":\"foundation.electrical.electrical\"},{\"id\":\"b\",\"label\":\"b\",\"type\":\"foundation.electrical.electrical\"},{\"id\":\"c\",\"label\":\"c\",\"type\":\"foundation.electrical.electrical\"}],\"Right\":[{\"id\":\"R\",\"label\":\"R\",\"type\":\"foundation.mechanical.rotational.rotational\"},{\"id\":\"C\",\"label\":\"C\",\"type\":\"foundation.mechanical.rotational.rotational\"}],\"Top\":[]}"
  Scope : Scope  NumInputPorts=4
      settings: ActiveDisplayYMinimum=-2500.2768341970282  ActiveDisplayYMaximum=2500.1048598569782
  Simulink-PS Converter1 : nesl_utility/Simulink-PS Converter  PhysicalDomain=network_engine_domain  SubClassName=ps_input  LeftPortType=input  RightPortType=output  PseudoPeriodic=off  Frequencies=[]  NoiseDistribution=none  NoiseParameters=[]  Unit=1  AffineConversion=off  FilteringAndDerivatives=provide  SimscapeFilterOrder=1  InputFilterTimeConstant=1e-6  UdotUserProvided=0
  Simulink-PS Converter2 : nesl_utility/Simulink-PS Converter  PhysicalDomain=network_engine_domain  SubClassName=ps_input  LeftPortType=input  RightPortType=output  PseudoPeriodic=off  Frequencies=[]  NoiseDistribution=none  NoiseParameters=[]  Unit=1  AffineConversion=off  FilteringAndDerivatives=provide  SimscapeFilterOrder=1  InputFilterTimeConstant=1e-6  UdotUserProvided=0
  Simulink-PS Converter3 : nesl_utility/Simulink-PS Converter  PhysicalDomain=network_engine_domain  SubClassName=ps_input  LeftPortType=input  RightPortType=output  PseudoPeriodic=off  Frequencies=[]  NoiseDistribution=none  NoiseParameters=[]  Unit=1  AffineConversion=off  FilteringAndDerivatives=provide  SimscapeFilterOrder=1  InputFilterTimeConstant=1e-6  UdotUserProvided=0
  Solver Configuration : nesl_utility/Solver Configuration  PhysicalDomain=network_engine_domain  SubClassName=solver  LeftPortType=input  RightPortType=generic  Tones=[]  Harmonics=[]  SimulateNoise=off  Profile=off  UseLocalSampling=off  EnableSwitchedLinearOptims=on  FrequencyDomain=off  UseCCode=off  RelTol=0.001  AbsTol=1e-06  MinStep=1e-09  ToWorkspace=off  RevertToSquareIcSolve=off  NumHomotopyIterations=100  PhasorMode=off  PhasorModeNumHarmonics=1  ConsistencySolver=NEWTON_XTOL_AFTER_FTOL  IndexReductionMethod=DerivativeReplacement  DoDC=off  ResidualTolerance=1e-09  ConsistencyTolSource=GLOBAL  ConsistencyAbsTol=0.001  ConsistencyRelTol=0.001  ConsistencyTolFactor=0.001  UseLocalSolver=off  LocalSolverChoice=NE_BACKWARD_EULER_ADVANCER  ResolveIndetEquations=on  FunctionEvalNumThread=1  LocalSolverSampleTime=0.001  DoFixedCost=off  MaxNonlinIter=3  MaxModeIter=2  ComputeImpulses=off  ImpulseIterations=2  LinearAlgebra=Sparse  LinearAlgebraNumThread=0  EquationFormulation=NE_TIME_EF  DelaysMemoryBudget=1024  AutomaticFiltering=on  FilteringTimeConstant=0.001  PartitionStorageMethod=AS_NEEDED  PartitionMemoryBudget=1024  PartitionMethod=FAST  MultibodyUseLocalSolver=off  MultibodyLocalSolverChoice=ODE1  MultibodyLocalSolverSampleTime=0.001
  rads2rpm : Gain  Gain=60/(2*pi)
  MeasSigs : Outport  VectorParamsAs1DForOutWhenUnconnected=off
  wires:
  ElecSensor/1(Iabc) -> [Iabc]
  ElecSensor/2(Vabc) -> [Vabc]
  Demux/2 -> Simulink-PS Converter2/1
  Demux/1 -> Simulink-PS Converter1/1
  Demux/3 -> Simulink-PS Converter3/1
  MechSensor/1(wm) -> [wm]
  MechSensor/2(thm) -> [thetam]
  MechSensor/3(Tm) -> [Tm]
  [wm] -> Bus Creator/1  "wm"
  [Iabc] -> Bus Creator/2  "Iabc"
  [thetam] -> Bus Creator/3  "thetam"
  Bus Creator/1 -> MeasSigs/1
  MotCmds/1 -> Bus Selector/1
  Bus Selector/1 -> Demux/1  "<Vabc>"
  [wm] -> rads2rpm/1
  rads2rpm/1 -> Scope/1  "Nm"
  [Tm] -> Scope/2  "Tm"
  [Vabc] -> Scope/3  "Vabc"
  [Iabc] -> Scope/4  "Iabc"
  connections:
  Simulink-PS Converter2/RConn1 -- Controlled Voltage Source2/RConn1
  Simulink-PS Converter3/RConn1 -- Controlled Voltage Source3/RConn1
  ElecSensor/RConn3 -- Permanent Magnet Synchronous Motor/LConn3
  ElecSensor/LConn2 -- Controlled Voltage Source2/LConn1
  Controlled Voltage Source3/RConn2 -- Controlled Voltage Source1/RConn2 -- Controlled Voltage Source2/RConn2 -- ElecSensor/RConn4 -- Electrical Reference/LConn1
  ElecSensor/RConn2 -- Permanent Magnet Synchronous Motor/LConn2
  ElecSensor/RConn1 -- Permanent Magnet Synchronous Motor/LConn1
  ElecSensor/LConn3 -- Controlled Voltage Source3/LConn1
  ElecSensor/LConn1 -- Controlled Voltage Source1/LConn1
  Simulink-PS Converter1/RConn1 -- Controlled Voltage Source1/RConn1
  Permanent Magnet Synchronous Motor/RConn2 -- Solver Configuration/RConn1 -- Mechanical Rotational Reference/LConn1 -- MechSensor/LConn2
  MechSensor/RConn1 -- MechLoad/LConn1
  MechLoad/LConn2 -- MechSensor/RConn2
  MechSensor/LConn1 -- Permanent Magnet Synchronous Motor/RConn1

== system fix_Current_sync/Subsystem5/Controller ==
  TestSigs : Inport
  MeasSigs : Inport  Port=2
  DriverPeripherals : Subsystem
  FOC : Subsystem
  SensorPeripherals : Subsystem
  TestChannel : Subsystem
  MotCmds : Outport  VectorParamsAs1DForOutWhenUnconnected=off
  wires:
  FOC/1(Vabc) -> DriverPeripherals/1(Vabc)
  DriverPeripherals/1(MotCmds) -> MotCmds/1
  TestSigs/1 -> TestChannel/1(TestSigs)
  TestChannel/1(wmref) -> FOC/1(wmref)
  MeasSigs/1 -> SensorPeripherals/1(MeasSigs)
  SensorPeripherals/1(wm) -> FOC/2(wm)
  SensorPeripherals/2(Iabc) -> FOC/3(Iabc)
  SensorPeripherals/3(thetam) -> FOC/4(thetam)

== system fix_Current_sync/Subsystem5/Evaluation ==
  TestSigs : Inport
  MeasSigs : Inport  Port=2
  Bus Selector : BusSelector  OutputSignals=wmref
  Bus Selector1 : BusSelector  OutputSignals=wm,thetam
  Mux : Mux  Inputs=2
  Scope : Scope
      settings: ActiveDisplayYMinimum=-3107.1721459970354  ActiveDisplayYMaximum=3159.6442979714316
  rads2rpm : Gain
  Out1 : Outport
  wires:
  TestSigs/1 -> Bus Selector/1
  Mux/1 -> rads2rpm/1
  rads2rpm/1 -> Scope/1
  MeasSigs/1 -> Bus Selector1/1
  Bus Selector/1 -> Mux/1  "<wmref>"
  Bus Selector1/2 -> Out1/1  "<thetam>"
  Bus Selector1/1 -> Mux/2  "<wm>"
